simulink model "EMSLEVEL2"  (R2026a)
settings: Solver=FixedStepDiscrete  StopTime=3  FixedStep=5e-6
PostLoadFcn:
  | params_ems;
  | Ts = 5e-6;
  | cap = p.invACDC(p.P_lim);
InitFcn:
  | params_ems;
  | Ts=5e-6;
  | cap=p.invACDC(p.P_lim);
values from neighbouring files (symbols this model uses):
  p = evalin('base', 'p')    [make_figures.m]    (also in params_ems.m = struct())
undefined symbols (not defined in the file or in its folder): DiscIntNeverNeededParam
libraries: fl_lib x16, nesl_utility x12, ee_lib x5, simulink_extras x1
settings Model: Creator=Kratos  LastModifiedBy=Kratos

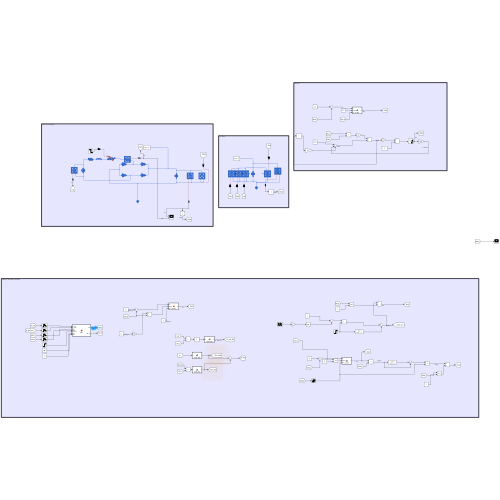
[thumbnail: Simulink's stored preview of the top-level diagram]
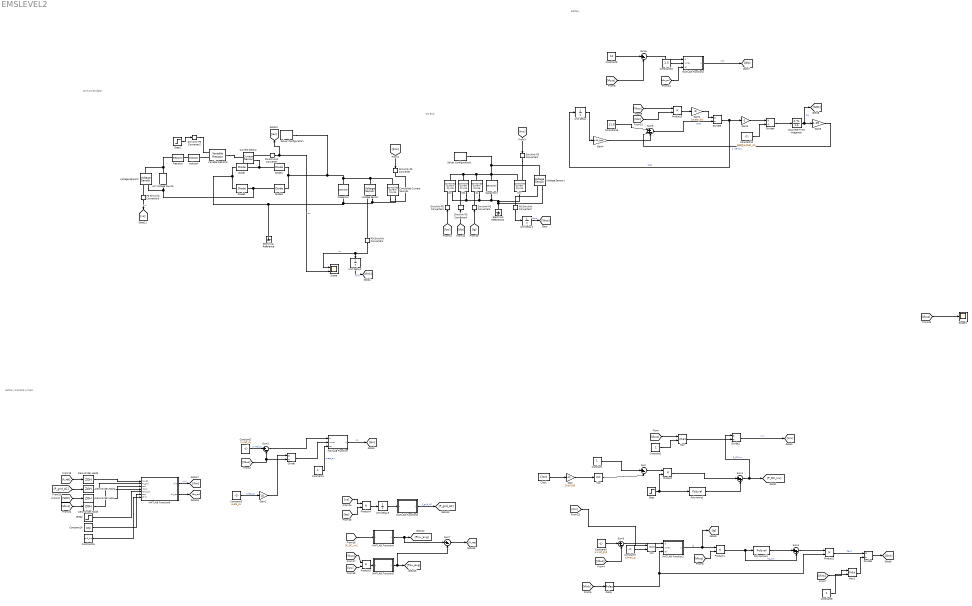
== system EMSLEVEL2 ==
  note: Battery and EMS system
  note: Battery
  note: Grid and Bridghe
  note: DC BUS
  AC Voltage Source : fl_lib/Electrical/Electrical Sources/AC Voltage Source  amp=p.Vgrid_pk V  shift=0 deg  frequency=50 Hz
  Capacitor : fl_lib/Electrical/Electrical Elements/Capacitor  c=p.C_link F  r=1e-6 Ohm  g=0 1/Ohm  i_specify=off  i_priority=None  i=0 A  i_nominal_specify=off  i_nominal_value=1  i_nominal_unit=A  v_specify=off  v_priority=None  v=0 V  v_nominal_specify=off  v_nominal_value=1  v_nominal_unit=V  vc_specify=off  vc_priority=High  vc=0 V  vc_nominal_specify=off  vc_nominal_value=1  vc_nominal_unit=V
  Capacitor1 : fl_lib/Electrical/Electrical Elements/Capacitor  c=p.C_bus F  r=1e-6 Ohm  g=0 1/Ohm  i_specify=off  i_priority=None  i=0 A  i_nominal_specify=off  i_nominal_value=1  i_nominal_unit=A  v_specify=on  v_priority=None  v=12.4 V  v_nominal_specify=off  v_nominal_value=1  v_nominal_unit=V  vc_specify=off  vc_priority=High  vc=0 V  vc_nominal_specify=off  vc_nominal_value=1  vc_nominal_unit=V
  Clock : simulink_extras/Flip Flops/Clock  period=2
  Constant{,1,4,8} (4 alike) : Constant
  Constant10 : Constant  Value=2.5
  Constant12 : Constant  Value=3600*p.Cbat_Ah
  Constant13 : Constant  Value=11.8
  Constant14 : Constant  Value=cap
  Constant15 : Constant  Value=p.P_lim
  Constant2 : Constant  Value=p.Vref_pv
  Constant3 : Constant  Value=p.eta_pv
  Constant5 : Constant  Value=p.Vref_grid
  Constant7 : Constant  Value=p.Imax_g
  Constant9 : Constant  Value=12
  Controlled Current Source1 : fl_lib/Electrical/Electrical Sources/Controlled Current Source
  Cos : Trigonometry  Operator=cos
  Current Sensor : fl_lib/Electrical/Electrical Sensors/Current Sensor
  Diode{,1..3} (4 alike) : ee_lib/Semiconductors & Converters/Diode  ModelType=ee.enum.diode.modelType.pwl  TableType=ee.enum.diode.tableType.IfMat  IfMat=[.07, .12, .19, 1.75, 4.24, 7.32, 11.2; .16, .3, .72, 2.14, 5.02, 8.35, 13.12] A  VfMat=[.9, 1.15, 1.25, 1.5, 1.75, 2.17, 2.6, 2.85; .58, .68, .75, 1.1, 1.38, 1.77, 2.27, 2.7] V  TjVec=[25, 125] degC  VfVec=[.5, .7, .9, 1.3, 1.7, 2.1, 2.5] V  IfVec=[.1, .2, .5, 1, 2, 4, 7, 10] A  IrMat=[1e-06, 2e-06, 5e-06, 1e-05, 2.5e-05, 5e-05, .0001; 2e-06, 5e-06, 1e-05, 4e-05, 8e-05, .0002, .0005] A  VrMat=[10, 100, 200, 250, 300, 325, 350; 10, 70, 160, 220, 270, 300, 320] V  VrVec=[10, 20, 40, 50, 70, 80, 100] V  IrVec=[1e-06, 2e-06, 5e-06, 1e-05, 2e-05, 5e-05, .0001] A  Vf=0.8 V  Ron=0.3 Ohm  Goff=1e-8 S  prmExp=ee.enum.diode.expParam.useTwo  I12=[.0137, .545] A  V12=[.6, .7] V  RS=0 Ohm  Tmeas=298.15 K  IS=1e-12 A  ec=1  I1=0.0137 A  V1=0.6 V  N_series=1  N_parallel=1  ZenerEnable=false  Rz=0.3 Ohm  BV=30 V  C_param=ee.enum.diode.capParam.fixed  CJ=0 pF  CJ0=5 pF  Vvec=[.1, 10, 100] V  Cvec=[3.5, 1, .4] pF  VJ=1 V  Mgrad=0.5  FC=0.5  Q_param=ee.enum.diode.recoveryParam.off  iRM=-7.15 A  iF=4 A  didt=-750 A/us  trr_factor=3  trr=115 ns  Qrr=150 nA*s  Vr=-600 V  Ls=150 nH  Erec=0.03 J  TT=50 ns  tau=100 ns  T_param=ee.enum.diode.temperatureParam.off  Tdevice=298.15 K  I1_T2=0.245 A  V1_T2=0.5 V  IS_T2=1.25e-7 A  Tmeas2=125 degC  XTI_param=ee.enum.diode.xtiParam.pn  XTI=3  EG_param=ee.enum.diode.egapParam.material_si  EG=1.11 eV  dBVdT=0 V/K  enable_fault_input=simscape.enum.onoff.off  i_specify=off  i_priority=None  i=0 A  i_nominal_specify=off  i_nominal_value=1  i_nominal_unit=A  v_specify=off  v_priority=None  v=0 V  v_nominal_specify=off  v_nominal_value=1  v_nominal_unit=V  v_capacitor_specify=off  v_capacitor_priority=None  v_capacitor=0 V  v_capacitor_nominal_specify=off  v_capacitor_nominal_value=1  v_capacitor_nominal_unit=V  Qj_specify=off  Qj_priority=High  Qj=0 C  Qj_nominal_specify=off  Qj_nominal_value=1  Qj_nominal_unit=C  i_diode_specify=off  i_diode_priority=None  i_diode=0 A  i_diode_nominal_specify=off  i_diode_nominal_value=1  i_diode_nominal_unit=A  v_diode_specify=off  v_diode_priority=None  v_diode=0 V  v_diode_nominal_specify=off  v_diode_nominal_value=1  v_diode_nominal_unit=V  i_capacitor_specify=off  i_capacitor_priority=None  i_capacitor=0 A  i_capacitor_nominal_specify=off  i_capacitor_nominal_value=1  i_capacitor_nominal_unit=A  fidelity_level=ee.enum.diode.fidelity.includeChargeDyn  rec_loss_model=ee.enum.diode.reverseRecoveryModelTabulateUpTo3D.fixed  ErecVal=0 J  scaleWithIandV=true  ErecMat=zeros(2, 3) J  ErecMat3D=zeros(2, 3, 2) J  TjrecVec=[298.15, 398.15] K  IfrecVec=[.1, 1, 10] A  IrecVal=10 A  VrecVal=10 V  VrecVec=[0, 100] V  tFilter=1 / 1000 / 100 s  thermal_network_parameterization=ee.enum.thermalNetworkTopology.junctionCase  Rth=[0, 10] K/W  Rth_Cauer=[1, 3, 10] K/W  Rth_Foster=[.08, .14, .22, .16] K/W  thermal_mass_parameterization=ee.enum.thermalNetwork.timeconstant  thermal_mass=[0, 1] J/K  thermal_mass_Cauer=[.1, .3, 1] J/K  thermal_mass_Foster=[.001, .005, .05, .5] J/K  thermal_time_constant=[0, 10] s  thermal_time_constant_Cauer=[1, 3, 10] s  thermal_time_constant_Foster=[7e-05, .0007, .01, .08] s  thermal_mass_initial_temperatures=[25, 25] degC  thermal_mass_initial_temperatures_Cauer=[25, 25, 25] degC  junction_thermal_mass=0.01 J/K  Tvec_initial_Foster=[25, 25, 25, 25] degC  no_thermal_network=0  junction_temperature_specify=off  junction_temperature_priority=None  junction_temperature=25 degC  junction_temperature_nominal_specify=off  junction_temperature_nominal_value=1  junction_temperature_nominal_unit=degC
  Discrete-Time Integrator : DiscreteIntegrator  InitialCondition=p.SOC0  SampleTime=Ts  LimitOutput=on  UpperSaturationLimit=1  LowerSaturationLimit=0  ICPrevOutput=DiscIntNeverNeededParam  ICPrevScaledInput=DiscIntNeverNeededParam
  Divide{,1..4} (5 alike) : Product  Inputs=*/
  Electrical Reference : fl_lib/Electrical/Electrical Elements/Electrical Reference
  Electrical Reference1 : fl_lib/Electrical/Electrical Elements/Electrical Reference
  Gain : Gain  Gain=2*pi*100
  Gain1 : Gain  Gain=10
  Gain2 : Gain  Gain=1/p.eta_dis
  Gain3 : Gain  Gain=-1
  Gain4 : Gain  Gain=p.R0_bat
  Gain5 : Gain  Gain=1.05
  Idis : fl_lib/Electrical/Electrical Sources/Controlled Current Source
  Ig : fl_lib/Electrical/Electrical Sources/Controlled Current Source
  Iinv : fl_lib/Electrical/Electrical Sources/Controlled Current Source
  Inductor : ee_lib/Passive/Inductor  l=p.L_src mH  enable_L_tol=ee.enum.toleranceApplication.none  L_tol=20  tol_distribution=ee.enum.toleranceDistribution.uniform  nSigma=4  r=0 Ohm  g=1e-9 1/Ohm  enable_operating_limits=ee.enum.enable.no  operating_limit_action=ee.enum.passive.reportOpLim.warn  max_working_current=1 A  power_rating=1 W  i_L_specify=off  i_L_priority=High  i_L=0 A  i_L_nominal_specify=off  i_L_nominal_value=1  i_L_nominal_unit=A
  Ipv : fl_lib/Electrical/Electrical Sources/Controlled Current Source
  MATLAB Function : MATLAB Function  TreatAsAtomicUnit=on
  MATLAB Function1 : MATLAB Function  TreatAsAtomicUnit=on
  MATLAB Function2 : MATLAB Function  TreatAsAtomicUnit=on
  MATLAB Function3 : MATLAB Function  TreatAsAtomicUnit=on
  MATLAB Function4 : MATLAB Function  TreatAsAtomicUnit=on
  MATLAB Function5 : MATLAB Function  TreatAsAtomicUnit=on
  MATLAB Function6 : MATLAB Function  TreatAsAtomicUnit=on
  Max : MinMax  Function=max  Inputs=2
  Max1 : MinMax  Function=max  Inputs=2
  Min : MinMax  Inputs=2
  PS-Simulink Converter{,1..3} (4 alike) : nesl_utility/PS-Simulink Converter  PhysicalDomain=network_engine_domain  SubClassName=ps_output  LeftPortType=input  RightPortType=output  PseudoPeriodic=off  Frequencies=[]  VectorFormat=inherit  Unit=inherit  AffineConversion=off
  Polynomial : Polyval  Coefs=[p.inv_k2 p.inv_k1 p.inv_P0]
  Polynomial1 : Polyval  Coefs=[p.fly_k2 p.fly_k1 p.fly_P0]
  Product{,1..5} (6 alike) : Product
  Relay : Relay  OnSwitchValue=200  OffSwitchValue=150
  Resistor : fl_lib/Electrical/Electrical Elements/Resistor  R=p.R_src Ohm  i_specify=off  i_priority=None  i=0 A  i_nominal_specify=off  i_nominal_value=1  i_nominal_unit=A  v_specify=off  v_priority=None  v=0 V  v_nominal_specify=off  v_nominal_value=1  v_nominal_unit=V
  Scope : Scope  NumInputPorts=2
      settings: ActiveDisplayYMinimum=170.24534351528209  ActiveDisplayYMaximum=357.03867982724347
  Scope1 : Scope
      settings: ActiveDisplayYMinimum=1.9466959018044792  ActiveDisplayYMaximum=13.161469029481562
  Simulink-PS Converter{,1..5} (6 alike) : nesl_utility/Simulink-PS Converter  PhysicalDomain=network_engine_domain  SubClassName=ps_input  LeftPortType=input  RightPortType=output  PseudoPeriodic=off  Frequencies=[]  NoiseDistribution=none  NoiseParameters=[]  Unit=1  AffineConversion=off  FilteringAndDerivatives=provide  SimscapeFilterOrder=1  InputFilterTimeConstant=0.001  UdotUserProvided=0
  Solver Configuration : nesl_utility/Solver Configuration  PhysicalDomain=network_engine_domain  SubClassName=solver  LeftPortType=input  RightPortType=generic  Tones=[]  Harmonics=[]  SimulateNoise=off  Profile=off  UseLocalSampling=off  EnableSwitchedLinearOptims=on  FrequencyDomain=off  UseCCode=off  RelTol=0.001  AbsTol=0.001  MinStep=1e-09  ToWorkspace=off  RevertToSquareIcSolve=off  NumHomotopyIterations=100  PhasorMode=off  PhasorModeNumHarmonics=1  ConsistencySolver=NEWTON_XTOL_AFTER_FTOL  CanonicalOrdering=CANONICAL  OptimizeIntermediates=OPTIMIZED  IndexReductionMethod=DerivativeReplacement  DoDC=off  ResidualTolerance=1e-09  ConsistencyTolSource=GLOBAL  ConsistencyAbsTol=0.001  ConsistencyRelTol=0.001  ConsistencyTolFactor=0.001  UseLocalSolver=on  LocalSolverChoice=NE_BACKWARD_EULER_ADVANCER  ResolveIndetEquations=on  FunctionEvalNumThread=1  LocalSolverSampleTime=Ts  DoFixedCost=off  MaxNonlinIter=3  MaxModeIter=2  ComputeImpulses=off  ImpulseIterations=2  LinearAlgebra=auto  LinearAlgebraNumThread=0  EquationFormulation=NE_TIME_EF  DelaysMemoryBudget=1024  AutomaticFiltering=on  FilteringTimeConstant=0.001  PartitionStorageMethod=AS_NEEDED  PartitionMemoryBudget=1024  PartitionMethod=ROBUST  MultibodyUseLocalSolver=off  MultibodyLocalSolverChoice=ODE1  MultibodyLocalSolverSampleTime=0.001
  Solver Configuration1 : nesl_utility/Solver Configuration  PhysicalDomain=network_engine_domain  SubClassName=solver  LeftPortType=input  RightPortType=generic  Tones=[]  Harmonics=[]  SimulateNoise=off  Profile=off  UseLocalSampling=off  EnableSwitchedLinearOptims=on  FrequencyDomain=off  UseCCode=off  RelTol=0.001  AbsTol=0.001  MinStep=1e-09  ToWorkspace=off  RevertToSquareIcSolve=off  NumHomotopyIterations=100  PhasorMode=off  PhasorModeNumHarmonics=1  ConsistencySolver=NEWTON_XTOL_AFTER_FTOL  CanonicalOrdering=CANONICAL  OptimizeIntermediates=OPTIMIZED  IndexReductionMethod=DerivativeReplacement  DoDC=off  ResidualTolerance=1e-09  ConsistencyTolSource=GLOBAL  ConsistencyAbsTol=0.001  ConsistencyRelTol=0.001  ConsistencyTolFactor=0.001  UseLocalSolver=on  LocalSolverChoice=NE_BACKWARD_EULER_ADVANCER  ResolveIndetEquations=on  FunctionEvalNumThread=1  LocalSolverSampleTime=Ts  DoFixedCost=off  MaxNonlinIter=3  MaxModeIter=2  ComputeImpulses=off  ImpulseIterations=2  LinearAlgebra=auto  LinearAlgebraNumThread=0  EquationFormulation=NE_TIME_EF  DelaysMemoryBudget=1024  AutomaticFiltering=on  FilteringTimeConstant=0.001  PartitionStorageMethod=AS_NEEDED  PartitionMemoryBudget=1024  PartitionMethod=ROBUST  MultibodyUseLocalSolver=off  MultibodyLocalSolverChoice=ODE1  MultibodyLocalSolverSampleTime=0.001
  Step : Step  Time=0.8  InitialValue=20  FinalValue=40  SampleTime=0
  Step1 : Step  Time=0.15  InitialValue=10  FinalValue=0.001  SampleTime=0
  Step2 : Step  Time=1.5  SampleTime=0
  Sum{,2..3,5,7} (5 alike) : Sum  Inputs=|+-
  Sum1 : Sum  Inputs=|++
  Sum4 : Sum  Inputs=|++
  Sum6 : Sum  Inputs=|++-
  Unit Delay : UnitDelay  SampleTime=Ts
  Unit Delay1 : UnitDelay  InitialCondition=12.4  SampleTime=Ts
  Unit Delay2 : UnitDelay  SampleTime=Ts
  Unit Delay3 : UnitDelay  SampleTime=Ts
  Variable Resistor : fl_lib/Electrical/Electrical Elements/Variable Resistor  Rmin=0 Ohm  thermalEnable=false  thermal_mass=1 J/K  i_specify=off  i_priority=None  i=0 A  i_nominal_specify=off  i_nominal_value=1  i_nominal_unit=A  v_specify=off  v_priority=None  v=0 V  v_nominal_specify=off  v_nominal_value=1  v_nominal_unit=V  T_specify=off  T_priority=None  T=300 K  T_nominal_specify=off  T_nominal_value=1  T_nominal_unit=K
  Voltage Sensor : fl_lib/Electrical/Electrical Sensors/Voltage Sensor
  Voltage Sensor1 : fl_lib/Electrical/Electrical Sensors/Voltage Sensor
  Voltage Sensor2 : fl_lib/Electrical/Electrical Sensors/Voltage Sensor
  Zero-Order Hold{,1..3} (4 alike) : ZeroOrderHold  SampleTime=0.1
  wires:
  PS-Simulink Converter/1 -> [iac], Scope/2  "iac"
  PS-Simulink Converter1/1 -> Unit Delay2/1, Scope/1  "Vc"
  PS-Simulink Converter2/1 -> Unit Delay1/1
  Clock/1 -> Gain/1
  Gain/1 -> Cos/1
  Constant/1 -> Sum/1
  Cos/1 -> Sum/2
  Sum/1 -> Product/1
  Step/1 -> Product/2, Polynomial/1
  Polynomial/1 -> Sum1/2
  Product/1 -> Sum1/1
  Sum1/1 -> Divide1/1, [P_DC_inv]  "P_DC,inv"
  [Vbus] -> Max/1
  Constant1/1 -> Max/2
  Max/1 -> Divide1/2
  Divide1/1 -> [iinv]  "iinv"
  [Ilink] -> Simulink-PS Converter/1
  Constant2/1 -> Sum2/1  "p.Vref_pv"
  [Vbus] -> Sum2/2, Divide/2
  Sum2/1 -> MATLAB Function/1(e)
  Constant3/1 -> Gain1/1  "p.eta_pv"
  Gain1/1 -> Divide/1
  Divide/1 -> MATLAB Function/2(umax)
  Constant4/1 -> MATLAB Function/3(en)  "p.eta_pv"
  MATLAB Function/1(u) -> [Ipv]  "ipv"
  [iinv] -> Simulink-PS Converter1/1
  Step1/1 -> Simulink-PS Converter2/1
  Constant5/1 -> Sum3/1
  [Vbus] -> Sum3/2
  [ilim] -> Min/1
  Sum3/1 -> MATLAB Function1/1(e)
  Min/1 -> MATLAB Function1/2(umax)
  Constant7/1 -> Min/2
  MATLAB Function1/1(u) -> [Ig], Product1/1  "ig"
  [Vlink] -> Relay/1
  Relay/1 -> Product2/2, MATLAB Function1/3(en)
  [Vbus] -> Product1/2
  Product1/1 -> Sum4/2, Polynomial1/1  "Pg_out"
  Polynomial1/1 -> Sum4/1
  Sum4/1 -> Product2/1
  Product2/1 -> Divide2/1  "Pg_in"
  [Vlink] -> Max1/1
  Constant8/1 -> Max1/2
  Max1/1 -> Divide2/2
  Divide2/1 -> [Ilink]
  Constant9/1 -> Sum5/1
  [Vbus] -> Sum5/2
  Sum5/1 -> MATLAB Function2/1(e)
  Constant10/1 -> MATLAB Function2/2(umax)
  MATLAB Function2/1(u) -> [Idis]  "idis"
  Gain2/1 -> Divide3/1
  [Idis] -> Product3/2
  [Vbus] -> Product3/1
  Divide3/1 -> Unit Delay/1, Gain3/1  "Ibat"
  Gain3/1 -> Divide4/1
  Constant12/1 -> Divide4/2
  Divide4/1 -> Discrete-Time Integrator/1
  Constant13/1 -> Sum6/1
  Unit Delay/1 -> Gain4/1
  Gain4/1 -> Sum6/3
  Discrete-Time Integrator/1 -> [SOC], Gain5/1  "soc"
  Gain5/1 -> Sum6/2  "1..05*soc"
  [Ipv] -> Simulink-PS Converter3/1
  [Idis] -> Simulink-PS Converter4/1
  [Ig] -> Simulink-PS Converter5/1
  Product3/1 -> Gain2/1
  Sum6/1 -> Divide3/2  "Vbat"
  PS-Simulink Converter3/1 -> [vs]  "vs"
  [vs] -> Product4/1
  [iac] -> Product4/2
  MATLAB Function3/1(y) -> [P_grid_AC]  "P_grid_AC"
  [P_DC_inv] -> MATLAB Function4/1(u)
  MATLAB Function4/1(y) -> Sum7/1, [Pinv_avg]
  Product5/1 -> MATLAB Function5/1(u)
  [Vbus] -> Product5/1
  [Ipv] -> Product5/2
  MATLAB Function5/1(y) -> Sum7/2, [Ppv_avg]
  Sum7/1 -> [P_net]
  Zero-Order Hold/1 -> MATLAB Function6/3(soc)
  [P_net] -> Zero-Order Hold2/1
  [P_grid_AC] -> Zero-Order Hold1/1
  [SOC] -> Zero-Order Hold/1
  [Vbus] -> Zero-Order Hold3/1
  Zero-Order Hold3/1 -> MATLAB Function6/4(Vbus)
  Zero-Order Hold1/1 -> MATLAB Function6/2(P_grid)
  Zero-Order Hold2/1 -> MATLAB Function6/1(P_net)
  Step2/1 -> MATLAB Function6/5(ems_on)
  Constant14/1 -> MATLAB Function6/6(cap)
  Constant15/1 -> MATLAB Function6/7(Plim)
  MATLAB Function6/1(Ilim) -> [ilim]  "Ilim"
  MATLAB Function6/2(dis_en) -> [dis_en]
  [dis_en] -> MATLAB Function2/3(en)
  Unit Delay1/1 -> [Vbus]  "Vbus"
  Unit Delay2/1 -> [Vlink]  "Vlink"
  Product4/1 -> Unit Delay3/1
  Unit Delay3/1 -> MATLAB Function3/1(u)
  [Vbus] -> Scope1/1
  connections:
  Inductor/LConn1 -- Resistor/RConn1
  AC Voltage Source/LConn1 -- Voltage Sensor2/LConn1 -- Resistor/LConn1
  Diode1/LConn1 -- Current Sensor/RConn2 -- Diode/RConn1
  Diode3/LConn1 -- Voltage Sensor2/RConn2 -- AC Voltage Source/RConn1 -- Diode2/RConn1
  Diode/LConn1 -- Diode2/LConn1 -- Electrical Reference/LConn1 -- Controlled Current Source1/RConn2 -- Voltage Sensor/RConn2 -- Capacitor/RConn1
  Diode1/RConn1 -- Solver Configuration/RConn1 -- Controlled Current Source1/LConn1 -- Voltage Sensor/LConn1 -- Capacitor/LConn1 -- Diode3/RConn1
  PS-Simulink Converter/LConn1 -- Current Sensor/RConn1
  PS-Simulink Converter1/LConn1 -- Voltage Sensor/RConn1
  Solver Configuration1/RConn1 -- Ipv/LConn1 -- Idis/LConn1 -- Ig/LConn1 -- Iinv/RConn2 -- Capacitor1/LConn1 -- Voltage Sensor1/LConn1
  Capacitor1/RConn1 -- Ig/RConn2 -- Idis/RConn2 -- Ipv/RConn2 -- Iinv/LConn1 -- Voltage Sensor1/RConn2 -- Electrical Reference1/LConn1
  PS-Simulink Converter2/LConn1 -- Voltage Sensor1/RConn1
  Controlled Current Source1/RConn1 -- Simulink-PS Converter/RConn1
  Simulink-PS Converter1/RConn1 -- Iinv/RConn1
  Variable Resistor/LConn2 -- Inductor/RConn1
  Variable Resistor/RConn1 -- Current Sensor/LConn1
  Simulink-PS Converter2/RConn1 -- Variable Resistor/LConn1
  Simulink-PS Converter3/RConn1 -- Ipv/RConn1
  Simulink-PS Converter4/RConn1 -- Idis/RConn1
  Simulink-PS Converter5/RConn1 -- Ig/RConn1
  PS-Simulink Converter3/LConn1 -- Voltage Sensor2/RConn1

== matlab function EMSLEVEL2/MATLAB Function1 ==
  data: e input; u output; umax input; en input
function u = pi_ctrl(e, umax, en)
Kp = 2; Ki = 40; dt = 5e-6;
persistent x
if isempty(x), x = 0; end
if en < 0.5, x = 0; u = 0; return; end
u_raw = Kp*e + x;
u = min(max(u_raw,0), umax);
if u == u_raw || (u_raw > umax && e < 0) || (u_raw < 0 && e > 0)
    x = x + Ki*e*dt;
end
x = min(max(x,-umax), umax);
end

== matlab function EMSLEVEL2/MATLAB Function ==
  data: e input; u output; umax input; en input
function u = pi_ctrl(e, umax, en)
Kp = 2; Ki = 40; dt = 5e-6;
persistent x
if isempty(x), x = 0; end
if en < 0.5, x = 0; u = 0; return; end
u_raw = Kp*e + x;
u = min(max(u_raw,0), umax);
if u == u_raw || (u_raw > umax && e < 0) || (u_raw < 0 && e > 0)
    x = x + Ki*e*dt;
end
x = min(max(x,-umax), umax);
end

== matlab function EMSLEVEL2/MATLAB Function2 ==
  data: e input; u output; umax input; en input
function u = pi_ctrl(e, umax, en)
Kp = 2; Ki = 40; dt = 5e-6;
persistent x
if isempty(x), x = 0; end
if en < 0.5, x = 0; u = 0; return; end
u_raw = Kp*e + x;
u = min(max(u_raw,0), umax);
if u == u_raw || (u_raw > umax && e < 0) || (u_raw < 0 && e > 0)
    x = x + Ki*e*dt;
end
x = min(max(x,-umax), umax);
end

== matlab function EMSLEVEL2/MATLAB Function3 ==
  data: u input; y output
function y = cycle_avg(u)
N = 4000;                      % 20 ms / 5 us
persistent acc k last
if isempty(acc), acc = 0; k = 0; last = 0; end
acc = acc + u; k = k + 1;
if k == N, last = acc/N; acc = 0; k = 0; end
y = last;
end

== matlab function EMSLEVEL2/MATLAB Function4 ==
  data: u input; y output
function y = cycle_avg(u)
N = 4000;                      % 20 ms / 5 us
persistent acc k last
if isempty(acc), acc = 0; k = 0; last = 0; end
acc = acc + u; k = k + 1;
if k == N, last = acc/N; acc = 0; k = 0; end
y = last;
end

== matlab function EMSLEVEL2/MATLAB Function5 ==
  data: u input; y output
function y = cycle_avg(u)
N = 4000;                      % 20 ms / 5 us
persistent acc k last
if isempty(acc), acc = 0; k = 0; last = 0; end
acc = acc + u; k = k + 1;
if k == N, last = acc/N; acc = 0; k = 0; end
y = last;
end

== matlab function EMSLEVEL2/MATLAB Function6 ==
  data: P_net input; Ilim output; P_grid input; soc input; Vbus input; ems_on input; cap input; Plim input; dis_en output
function [Ilim, dis_en] = ems(P_net, P_grid, soc, Vbus, ems_on, cap, Plim)
Imax = 4.8; Kems = 0.2; T = 0.1;
persistent mode dis_ok Ilim_s
if isempty(mode), mode = 0; dis_ok = true; Ilim_s = Imax; end
if ems_on > 0.5
    if soc <= 0.40, dis_ok = false; end
    if soc >= 0.43, dis_ok = true;  end
    if P_net > cap && dis_ok
        if mode ~= 2
            mode = 2; Ilim_s = cap/max(Vbus,1);
        else
            Ilim_s = Ilim_s + Kems*(Plim - P_grid)*T;
        end
        Ilim_s = min(max(Ilim_s,0), Imax);
    else
        mode = 0; Ilim_s = Imax;
    end
end
Ilim = Ilim_s; dis_en = double(mode == 2);
end
